simulink model "F16_6DOF_R2024b"  (R2024b)
settings: Solver=VariableStepAuto  StartTime=0.0  StopTime=10.0  RelTol=1e-3
values from neighbouring files (symbols this model uses):
  AeroBP = f16_AerodynamicData.BP    [init_F16.m]
  AeroData = f16_AerodynamicData.data    [init_F16.m]
  b = 30.0 * ft2m    (= 9.144)    [init_F16.m]    (also in trim_F16.m = sin(phi)*sin(beta) + cos(phi)*sin(alpha)*cos(beta))
  cbar = 11.32 * ft2m    (= 3.450336)    [init_F16.m]
  dP_BP = [-100, 25, 50, 100]    [init_F16.m]
  EngBP = f16_EngineData.BP    [init_F16.m]
  EngData = f16_EngineData.data.Thrust_lbs    [init_F16.m]
  Euler_0 = [0;0;0]    [init_F16.m]
  ft2m = 0.3048    [init_F16.m]
  gamma_R_SI = 1.4 * 1716.3 * R_conv    (= 401.812708631)    [init_F16.m]
  h_trop_SI = 35000 * ft2m    (= 10668)    [init_F16.m]
  He = 160.0 * slugft2_to_kgm2    (= 216.930890496)    [init_F16.m]
  I_mat = [ Ixx,  0,   -Ixz ... (first row only)    [init_F16.m]
  inv_I = inv(I_mat)    [init_F16.m]
  inv_tauT_tab = [1.0, 1.0, 0.1, 0.1]    [init_F16.m]
  lapse_SI = 0.703e-5 / ft2m    (= 2.30643044619e-05)    [init_F16.m]
  lbf2N = 4.448222    [init_F16.m]
  m = Weight / g    (= 9298.64438927)    [init_F16.m]
  omega_0 = [0;0;0]    [init_F16.m]
  P1_tab = [0, 50, 100]    [init_F16.m]
  P3_0 = 0    [init_F16.m]    (also in test_thrust_table2.m = interp1(thr_BP, P1_tab, cases(i,3)))
  Pos_0 = [0;0;-3048]    [init_F16.m]
  R0_SI = 2.377e-3 * (slug2kg / ft2m^3)    (= 1.22505555728)    [init_F16.m]
  R_ps_SI = 1715 * R_conv    (= 286.79168448)    [init_F16.m]
  S = 300.0 * (ft2m^2)    (= 27.870912)    [init_F16.m]
  T0_SI = 519.0 / 1.8    (= 288.333333333)    [init_F16.m]
  T_iso_SI = 390 / 1.8    (= 216.666666667)    [init_F16.m]
  thr_BP = [0, 77, 100]    [init_F16.m]
  V_body_0 = [131.28; 0; 0]    [init_F16.m]
  Weight = 20500.0 * lbf2N    (= 91188.551)    [init_F16.m]
  xcg = 0.35    [init_F16.m]
  xcgr = 0.35    [init_F16.m]
libraries: simulink_extras x2
(part 1 of 2)
settings Model: Creator=dilan  LastModifiedBy=emirh

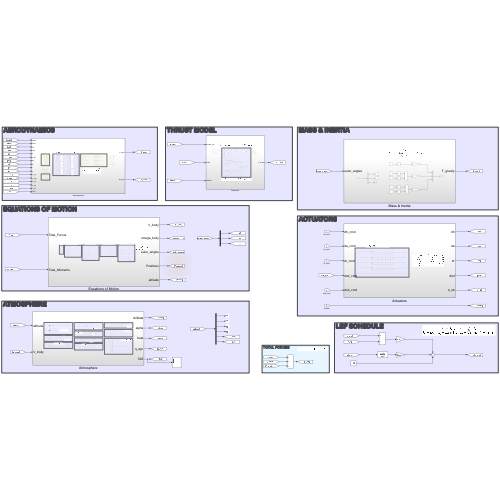
[thumbnail: Simulink's stored preview of the top-level diagram]
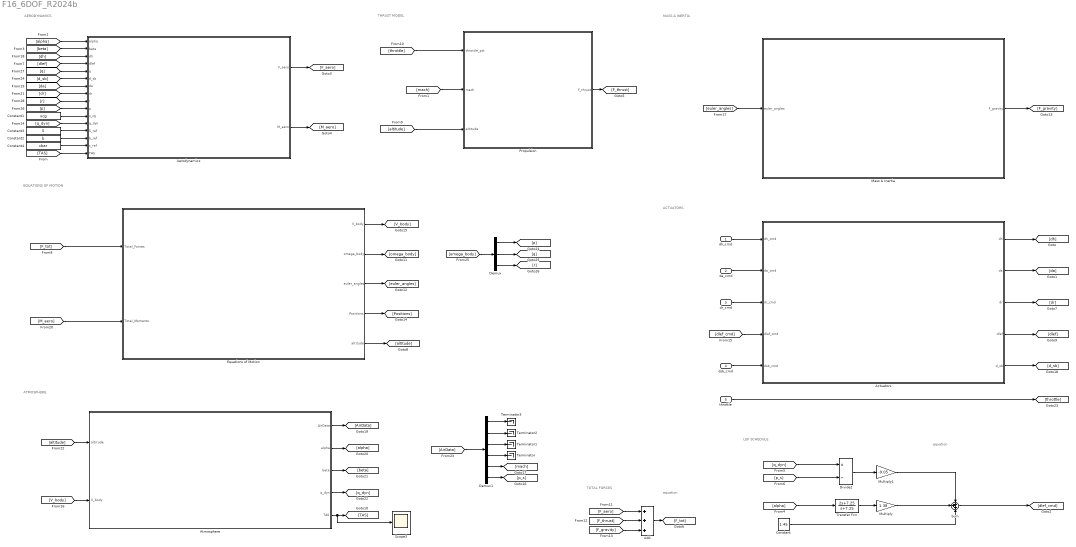
== system F16_6DOF_R2024b ==
  note: TOTAL FORCES
  note: THRUST MODEL
  note: AERODYNAMICS
  note: LEF SCHEDULE
  note: ATMOSPHERE
  note: ACTUATORS
  note: MASS & INERTIA
  note: EQUATIONS OF MOTION
  note: equation
  note: equation
  dh_cmd : Inport
  da_cmd : Inport  Port=2
  dr_cmd : Inport  Port=3
  dsb_cmd : Inport  Port=4
  throttle : Inport  Port=5
  Actuators : Subsystem
  Add : Sum  Inputs=+++
  Aerodynamics : Subsystem
  Atmosphere : Subsystem
  Constant : Constant  Value=1.45
  Constant1 : Constant  Value=xcg
  Constant2 : Constant  Value=b
  Constant3 : Constant  Value=S
  Constant4 : Constant  Value=cbar
  Demux : Demux  Outputs=3
  Demux1 : Demux  Outputs=6
  Divide2 : Product  Inputs=*/
  Equations of Motion : Subsystem
  Mass & Inertia : Subsystem
  Multiply : Gain  Gain=1.38
  Multiply1 : Gain  Gain=-9.05
  Propulsion : Subsystem
  Scope3 : Scope
  Sum : Sum  Inputs=+++
  Terminator{,1..3} (4 alike) : Terminator
  Transfer Fcn : TransferFcn  Numerator=[2 7.25]  Denominator=[1 7.25]
  wires:
  [alpha] -> Aerodynamics/1(alpha)
  [beta] -> Aerodynamics/2(beta)
  Constant/1 -> Sum/3
  Multiply/1 -> Sum/2
  Multiply1/1 -> Sum/1
  Divide2/1 -> Multiply1/1
  Transfer Fcn/1 -> Multiply/1
  [alpha] -> Transfer Fcn/1
  [q_dyn] -> Divide2/1
  [p_s] -> Divide2/2
  [dlef] -> Aerodynamics/4(dlef)
  Aerodynamics/1(F_aero) -> [F_aero]
  Aerodynamics/2(M_aero) -> [M_aero]
  [altitude] -> Propulsion/3(altitude)
  [throttle] -> Propulsion/1(throttle_pct)
  Propulsion/1(F_thrust) -> [F_thrust]
  [F_aero] -> Add/1
  [F_thrust] -> Add/2
  [F_gravity] -> Add/3
  Add/1 -> [F_tot]
  [mach] -> Propulsion/2(mach)
  [q_dyn] -> Aerodynamics/12(q_dyn)
  [altitude] -> Atmosphere/1(altitude)
  [V_body] -> Atmosphere/2(V_body)
  Atmosphere/1(AirData) -> [AirData]
  Atmosphere/2(alpha) -> [alpha]
  Atmosphere/3(beta) -> [beta]
  Atmosphere/4(q_dyn) -> [q_dyn]
  Atmosphere/5(TAS) -> [TAS], Scope3/1
  [AirData] -> Demux1/1
  Demux1/1 -> Terminator3/1
  Demux1/2 -> Terminator2/1
  Demux1/3 -> Terminator1/1
  Demux1/4 -> Terminator/1
  Demux1/5 -> [mach]
  Demux1/6 -> [p_s]
  Sum/1 -> [dlef_cmd]
  dh_cmd/1 -> Actuators/1(dh_cmd)
  Actuators/1(dh) -> [dh]
  da_cmd/1 -> Actuators/2(da_cmd)
  Actuators/2(da) -> [da]
  dr_cmd/1 -> Actuators/3(dr_cmd)
  Actuators/3(dr) -> [dr]
  [dlef_cmd] -> Actuators/4(dlef_cmd)
  Actuators/4(dlef) -> [dlef]
  dsb_cmd/1 -> Actuators/5(dsb_cmd)
  Actuators/5(d_sb) -> [d_sb]
  throttle/1 -> [throttle]
  [dh] -> Aerodynamics/3(dh)
  [da] -> Aerodynamics/7(da)
  [dr] -> Aerodynamics/8(dr)
  [d_sb] -> Aerodynamics/6(d_sb)
  [TAS] -> Aerodynamics/16(TAS)
  [p] -> Aerodynamics/10(p)
  [q] -> Aerodynamics/5(q)
  [r] -> Aerodynamics/9(r)
  Constant1/1 -> Aerodynamics/11(x_cg)
  Constant3/1 -> Aerodynamics/13(S_ref)
  Constant2/1 -> Aerodynamics/14(b_ref)
  Constant4/1 -> Aerodynamics/15(c_ref)
  [euler_angles] -> Mass & Inertia/1(euler_angles)
  Mass & Inertia/1(F_gravity) -> [F_gravity]
  [F_tot] -> Equations of Motion/1(Total_Forces)
  [M_aero] -> Equations of Motion/2(Total_Moments)
  Equations of Motion/1(V_body) -> [V_body]
  Equations of Motion/2(omega_body) -> [omega_body]
  Equations of Motion/3(euler_angles) -> [euler_angles]
  Equations of Motion/4(Positions) -> [Positions]
  Equations of Motion/5(altitude) -> [altitude]
  [omega_body] -> Demux/1
  Demux/1 -> [p]
  Demux/2 -> [q]
  Demux/3 -> [r]

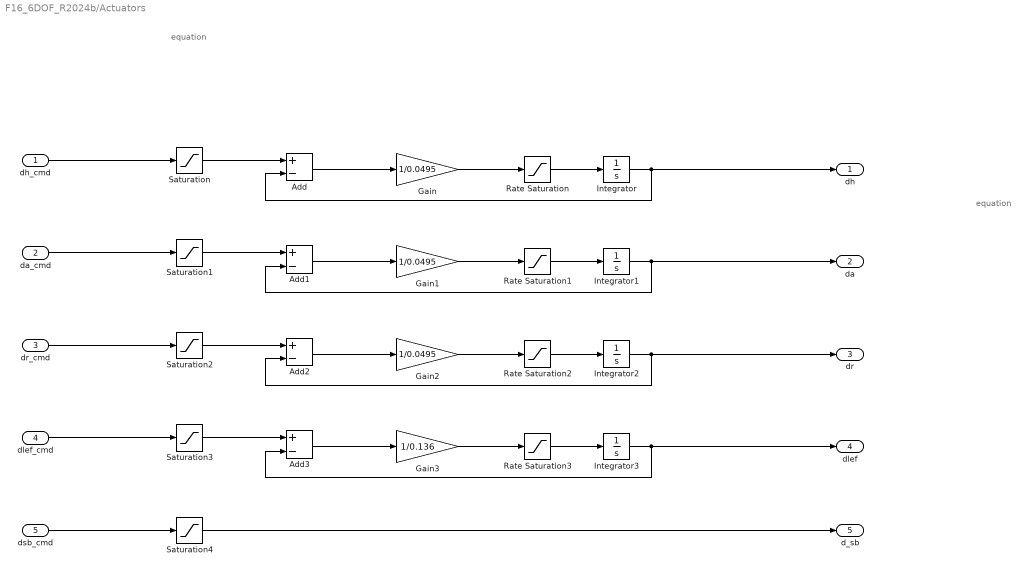
== system F16_6DOF_R2024b/Actuators ==
  note: equation
  note: equation
  dh_cmd : Inport
  da_cmd : Inport  Port=2
  dr_cmd : Inport  Port=3
  dlef_cmd : Inport  Port=4
  dsb_cmd : Inport  Port=5
  Add{,1..3} (4 alike) : Sum  Inputs=+-
  Gain : Gain  Gain=1/0.0495
  Gain1 : Gain  Gain=1/0.0495
  Gain2 : Gain  Gain=1/0.0495
  Gain3 : Gain  Gain=1/0.136
  Integrator{,1..3} (4 alike) : Integrator
  Rate Saturation : Saturate  UpperLimit=60  LowerLimit=-60
  Rate Saturation1 : Saturate  UpperLimit=80  LowerLimit=-80
  Rate Saturation2 : Saturate  UpperLimit=120  LowerLimit=-120
  Rate Saturation3 : Saturate  UpperLimit=25  LowerLimit=-25
  Saturation : Saturate  UpperLimit=25  LowerLimit=-25
  Saturation1 : Saturate  UpperLimit=21.5  LowerLimit=-21.5
  Saturation2 : Saturate  UpperLimit=30  LowerLimit=-30
  Saturation3 : Saturate  UpperLimit=25  LowerLimit=0
  Saturation4 : Saturate  UpperLimit=60  LowerLimit=0
  dh : Outport
  da : Outport  Port=2
  dr : Outport  Port=3
  dlef : Outport  Port=4
  d_sb : Outport  Port=5
  wires:
  dh_cmd/1 -> Saturation/1
  da_cmd/1 -> Saturation1/1
  dr_cmd/1 -> Saturation2/1
  dlef_cmd/1 -> Saturation3/1
  dsb_cmd/1 -> Saturation4/1
  Saturation/1 -> Add/1
  Add/1 -> Gain/1
  Gain/1 -> Rate Saturation/1
  Rate Saturation/1 -> Integrator/1
  Integrator/1 -> dh/1, Add/2
  Integrator1/1 -> da/1, Add1/2
  Rate Saturation1/1 -> Integrator1/1
  Gain1/1 -> Rate Saturation1/1
  Add1/1 -> Gain1/1
  Saturation1/1 -> Add1/1
  Add2/1 -> Gain2/1
  Gain2/1 -> Rate Saturation2/1
  Rate Saturation2/1 -> Integrator2/1
  Integrator2/1 -> dr/1, Add2/2
  Integrator3/1 -> dlef/1, Add3/2
  Rate Saturation3/1 -> Integrator3/1
  Gain3/1 -> Rate Saturation3/1
  Add3/1 -> Gain3/1
  Saturation4/1 -> d_sb/1
  Saturation2/1 -> Add2/1
  Saturation3/1 -> Add3/1

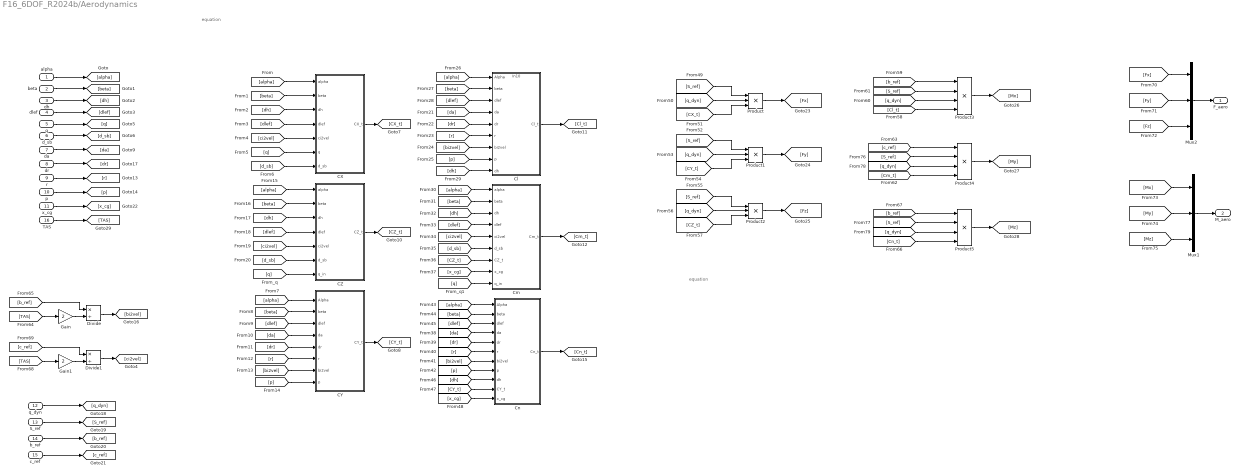
== system F16_6DOF_R2024b/Aerodynamics ==
  note: equation
  note: equation
  alpha : Inport
  beta : Inport  Port=2
  dh : Inport  Port=3
  dlef : Inport  Port=4
  q : Inport  Port=5
  d_sb : Inport  Port=6
  da : Inport  Port=7
  dr : Inport  Port=8
  r : Inport  Port=9
  p : Inport  Port=10
  x_cg : Inport  Port=11
  q_dyn : Inport  Port=12
  S_ref : Inport  Port=13
  b_ref : Inport  Port=14
  c_ref : Inport  Port=15
  TAS : Inport  Port=16
  CX : Subsystem
  CY : Subsystem
  CZ : Subsystem
  Cl : Subsystem
      settings: PortSchema="{\"entries\":[{\"content\":{\"sides\":[{\"content\":{\"connectorIds\":[\"In1\",\"In2\",\"In3\",\"In4\",\"In5\",\"In6\",\"In7\",\"In8\",\"In9\"]},\"type\":\"ConnectorPlacement.EquallySpacedRectSide\",\"uuid\":\"21997383-d6a2-4283-9afe-3717b1097433\"},{\"content\":{\"connectorIds\":[\"Out1\"],\"side\":\"RIGHT\"},\"type\":\"ConnectorPlacement.EquallySpacedRectSide\",\"uuid\":\"dad54f1b-8e4a-4bdd-ae1b-a5d035dab541\"},{\"content\":{\"connectorIds\":[\"In10\"],\"side\":\"TOP\"},\"type\":\"ConnectorPlacement.EquallySpacedRectSide\",\"uuid\":\"167dcd83-ef9f-4972-849f-adf1f6d78b80\"}]},\"type\":\"ConnectorPlacement.EquallySpacedConnector\",\"uuid\":\"1257b268-e5da-46f6-bd8b-58a49b5f7559\"}],\"packageUris\":[\"http://schema.mathworks.com/mf0/Connector/R2020b\"],\"version\":\"1.0\"}"
  Cm : Subsystem
  Cn : Subsystem
  Divide : Product  Inputs=*/
  Divide1 : Product  Inputs=*/
  Gain : Gain  Gain=2
  Gain1 : Gain  Gain=2
  Mux1 : Mux  Inputs=3
  Mux2 : Mux  Inputs=3
  Product : Product  Inputs=3
  Product1 : Product  Inputs=3
  Product2 : Product  Inputs=3
  Product3 : Product  Inputs=4
  Product4 : Product  Inputs=4
  Product5 : Product  Inputs=4
  F_aero : Outport
  M_aero : Outport  Port=2
  wires:
  [c_ref] -> Product4/1
  [dlef] -> CZ/4(dlef)
  [r] -> CY/6(r)
  [beta] -> CY/2(beta)
  [d_sb] -> CX/7(d_sb)
  da/1 -> [da]
  CX/1(CX_t) -> [CX_t]
  q/1 -> [q]
  [dr] -> Cl/5(dr)
  [p] -> CY/8(p)
  dr/1 -> [dr]
  [q_dyn] -> Product3/3
  CZ/1(CZ_t) -> [CZ_t]
  [dr] -> Cn/5(dr)
  [bi2vel] -> Cn/7(bi2vel)
  [da] -> CY/4(da)
  [x_cg] -> Cn/11(x_cg)
  [ci2vel] -> CZ/5(ci2vel)
  Cn/1(Cn_t) -> [Cn_t]
  [alpha] -> CY/1(Alpha)
  CY/1(CY_t) -> [CY_t]
  [Cn_t] -> Product5/4
  [dr] -> CY/5(dr)
  [dlef] -> CY/3(dlef)
  [bi2vel] -> CY/7(bi2vel)
  [q] -> CX/6(q)
  [da] -> Cn/4(da)
  [da] -> Cl/4(da)
  [CY_t] -> Cn/10(CY_t)
  S_ref/1 -> [S_ref]
  [dh] -> Cm/3(dh)
  [My] -> Mux1/2
  [dlef] -> CX/4(dlef)
  p/1 -> [p]
  dh/1 -> [dh]
  alpha/1 -> [alpha]
  Product3/1 -> [Mx]
  [d_sb] -> Cm/6(d_sb)
  [beta] -> CZ/2(beta)
  [ci2vel] -> CX/5(ci2vel)
  beta/1 -> [beta]
  [alpha] -> CX/1(alpha)
  [S_ref] -> Product1/1
  [S_ref] -> Product3/2
  [bi2vel] -> Cl/7(bi2vel)
  [dh] -> CX/3(dh)
  [CZ_t] -> Product2/3
  x_cg/1 -> [x_cg]
  [dlef] -> Cn/3(dlef)
  [Mz] -> Mux1/3
  [dh] -> Cl/9(dh)
  dlef/1 -> [dlef]
  r/1 -> [r]
  d_sb/1 -> [d_sb]
  [beta] -> CX/2(beta)
  [p] -> Cn/8(p)
  b_ref/1 -> [b_ref]
  [dlef] -> Cl/3(dlef)
  [ci2vel] -> Cm/5(ci2vel)
  [r] -> Cl/6(r)
  [r] -> Cn/6(r)
  [p] -> Cl/8(p)
  [d_sb] -> CZ/6(d_sb)
  [dlef] -> Cm/4(dlef)
  Cl/1(Cl_t) -> [Cl_t]
  Product1/1 -> [Fy]
  [dh] -> CZ/3(dh)
  [alpha] -> CZ/1(alpha)
  Product5/1 -> [Mz]
  [b_ref] -> Product5/1
  [alpha] -> Cl/1(Alpha)
  [beta] -> Cl/2(beta)
  q_dyn/1 -> [q_dyn]
  [beta] -> Cm/2(beta)
  [alpha] -> Cm/1(alpha)
  [dh] -> Cn/9(dh)
  [Fx] -> Mux2/1
  [Cm_t] -> Product4/4
  Product4/1 -> [My]
  Cm/1(Cm_t) -> [Cm_t]
  Mux1/1 -> M_aero/1
  [Fz] -> Mux2/3
  Mux2/1 -> F_aero/1
  [Fy] -> Mux2/2
  [Mx] -> Mux1/1
  [beta] -> Cn/2(beta)
  [alpha] -> Cn/1(Alpha)
  c_ref/1 -> [c_ref]
  [Cl_t] -> Product3/4
  [b_ref] -> Product3/1
  [x_cg] -> Cm/8(x_cg)
  [CZ_t] -> Cm/7(CZ_t)
  [q_dyn] -> Product/2
  Product2/1 -> [Fz]
  [S_ref] -> Product/1
  [q_dyn] -> Product1/2
  Product/1 -> [Fx]
  [CX_t] -> Product/3
  [S_ref] -> Product2/1
  [CY_t] -> Product1/3
  [q_dyn] -> Product2/2
  TAS/1 -> [TAS]
  [TAS] -> Gain/1
  Gain/1 -> Divide/2
  [b_ref] -> Divide/1
  Divide/1 -> [bi2vel]
  [c_ref] -> Divide1/1
  Gain1/1 -> Divide1/2
  [TAS] -> Gain1/1
  Divide1/1 -> [ci2vel]
  [q] -> CZ/7(q_in)
  [q] -> Cm/9(q_in)
  [S_ref] -> Product4/2
  [S_ref] -> Product5/2
  [q_dyn] -> Product4/3
  [q_dyn] -> Product5/3

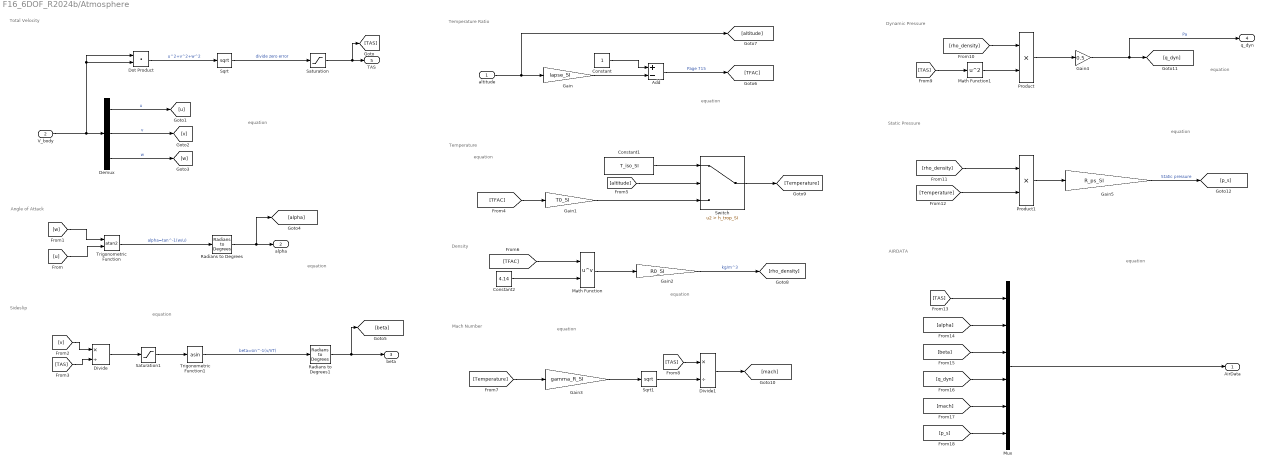
== system F16_6DOF_R2024b/Atmosphere ==
  note: AIRDATA
  note: Static Pressure
  note: Dynamic Pressure
  note: Mach Number
  note: Density
  note: Temperature
  note: Temperature Ratio
  note: Sideslip
  note: Angle of Attack
  note: Total Velocity
  note: equation
  note: equation
  note: equation
  note: equation
  note: equation
  note: equation
  note: equation
  note: equation
  note: equation
  note: equation
  altitude : Inport
  V_body : Inport  Port=2
  Add : Sum  Inputs=+-
  Constant : Constant
  Constant1 : Constant  Value=T_iso_SI
  Constant2 : Constant  Value=4.14
  Demux : Demux  Outputs=3
  Divide : Product  Inputs=*/
  Divide1 : Product  Inputs=*/
  Dot Product : DotProduct  OutDataTypeStr=Inherit: Inherit via internal rule
  Gain : Gain  Gain=lapse_SI
  Gain1 : Gain  Gain=T0_SI
  Gain2 : Gain  Gain=R0_SI
  Gain3 : Gain  Gain=gamma_R_SI
  Gain4 : Gain  Gain=0.5
  Gain5 : Gain  Gain=R_ps_SI
  Math Function : Math  Operator=pow
  Math Function1 : Math  Operator=square
  Mux : Mux  Inputs=6
  Product : Product
  Product1 : Product
  Radians to Degrees : simulink_extras/Transformations/Radians to Degrees
  Radians to Degrees1 : simulink_extras/Transformations/Radians to Degrees
  Saturation : Saturate  UpperLimit=inf  LowerLimit=0.1
  Saturation1 : Saturate  UpperLimit=1  LowerLimit=-1
  Sqrt : Sqrt
  Sqrt1 : Sqrt
  Switch : Switch  Criteria=u2 > Threshold  Threshold=h_trop_SI  SaturateOnIntegerOverflow=off  InputSameDT=off
  Trigonometric Function : Trigonometry  Operator=atan2
  Trigonometric Function1 : Trigonometry  Operator=asin
  AirData : Outport
  alpha : Outport  Port=2
  beta : Outport  Port=3
  q_dyn : Outport  Port=4
  TAS : Outport  Port=5
  wires:
  V_body/1 -> Dot Product/2, Dot Product/1, Demux/1
  altitude/1 -> [altitude], Gain/1
  Dot Product/1 -> Sqrt/1  "u^2+v^2+w^2"
  Demux/1 -> [u]  "u"
  Demux/2 -> [v]  "v"
  Demux/3 -> [w]  "w"
  Sqrt/1 -> Saturation/1  "divide zero error"
  Saturation/1 -> [TAS], TAS/1
  [w] -> Trigonometric Function/1
  [u] -> Trigonometric Function/2
  Trigonometric Function/1 -> Radians to Degrees/1  "alpha=tan^-1(w/u)"
  Radians to Degrees/1 -> [alpha], alpha/1
  [v] -> Divide/1
  [TAS] -> Divide/2
  Divide/1 -> Saturation1/1
  Saturation1/1 -> Trigonometric Function1/1
  Trigonometric Function1/1 -> Radians to Degrees1/1  "beta=sin^-1(v/VT)"
  Radians to Degrees1/1 -> [beta], beta/1
  Constant/1 -> Add/1
  Gain/1 -> Add/2
  Add/1 -> [TFAC]  "Page 715"
  [TFAC] -> Gain1/1
  Constant1/1 -> Switch/1
  [altitude] -> Switch/2
  Gain1/1 -> Switch/3
  [TFAC] -> Math Function/1
  Constant2/1 -> Math Function/2
  Math Function/1 -> Gain2/1
  Gain2/1 -> [rho_density]  "kg/m^3"
  Switch/1 -> [Temperature]
  [Temperature] -> Gain3/1
  Gain3/1 -> Sqrt1/1
  Sqrt1/1 -> Divide1/2
  [TAS] -> Divide1/1
  Divide1/1 -> [mach]
  [TAS] -> Math Function1/1
  [rho_density] -> Product/1
  Math Function1/1 -> Product/2
  Product/1 -> Gain4/1
  Gain4/1 -> q_dyn/1, [q_dyn]  "Pa"
  [rho_density] -> Product1/1
  [Temperature] -> Product1/2
  Product1/1 -> Gain5/1
  Gain5/1 -> [p_s]  "Static pressure"
  [TAS] -> Mux/1
  [alpha] -> Mux/2
  [beta] -> Mux/3
  [q_dyn] -> Mux/4
  [mach] -> Mux/5
  [p_s] -> Mux/6
  Mux/1 -> AirData/1

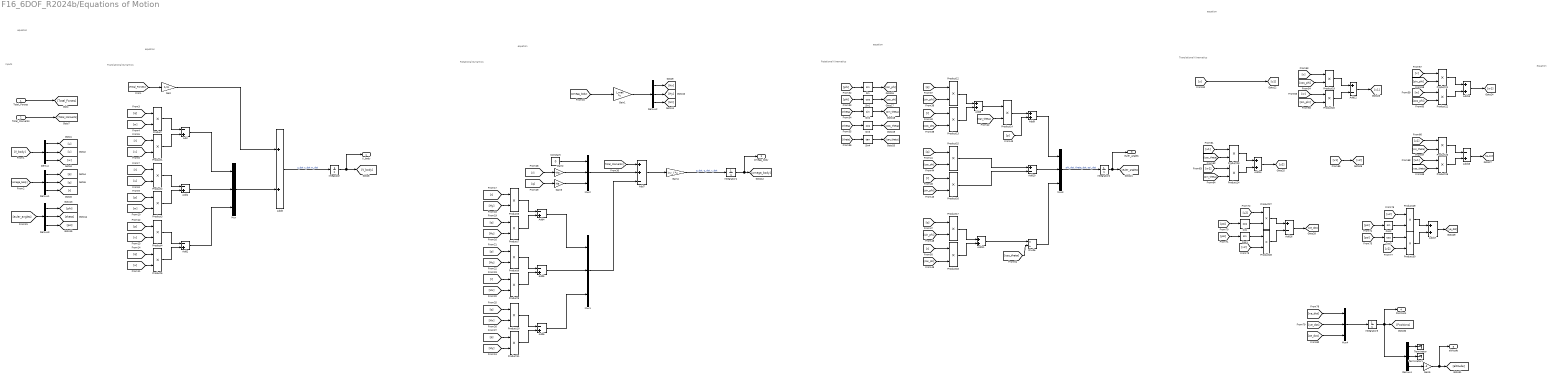
== system F16_6DOF_R2024b/Equations of Motion ==
  note: Inputs
  note: Translational Kinematics
  note: Rotational Kinematics
  note: Rotational Dynamics
  note: Translational Dynamics
  note: equation
  note: equation
  note: equation
  note: equation
  note: equation
  note: equation
  Total_Forces : Inport
  Total_Moments : Inport  Port=2
  Add{,1..2,4..6,15} (7 alike) : Sum  Inputs=-+
  Add10 : Sum  Inputs=+-
  Add{3,8..9,11,13..14,17} (7 alike) : Sum
  Add12 : Sum  Inputs=+-
  Add16 : Sum  Inputs=+-
  Add7 : Sum  Inputs=++-
  Constant : Constant  Value=0
  Cos : Trigonometry  Operator=cos
  Cos1 : Trigonometry
  Cos2 : Trigonometry
  Cos3 : Trigonometry  Operator=cos
  Demux{,1..4} (5 alike) : Demux  Outputs=3
  Divide : Product  Inputs=*/
  Gain : Gain  Gain=1/m
  Gain1 : Gain  Gain=I_mat  Multiplication=Matrix(K*u)
  Gain2 : Gain  Gain=-He
  Gain3 : Gain  Gain=He
  Gain4 : Gain  Gain=inv_I  Multiplication=Matrix(K*u)
  Gain5 : Gain  Gain=-1
  Integrator : Integrator  InitialCondition=V_body_0
  Integrator1 : Integrator  InitialCondition=omega_0
  Integrator2 : Integrator  InitialCondition=Euler_0
  Integrator3 : Integrator  InitialCondition=Pos_0
  Mux{,1..4} (5 alike) : Mux  Inputs=3
  Product{,1..30} (31 alike) : Product
  Sin : Trigonometry
  Sin1 : Trigonometry  Operator=cos
  Sin2 : Trigonometry
  Sin3 : Trigonometry  Operator=cos
  Sin4 : Trigonometry  Operator=tan
  Terminator : Terminator
  Terminator1 : Terminator
  V_body : Outport
  omega_body : Outport  Port=2
  euler_angles : Outport  Port=3
  Positions : Outport  Port=4
  altitude : Outport  Port=5
  wires:
  Total_Forces/1 -> [Total_Forces]
  [Total_Forces] -> Gain/1
  [V_body] -> Demux/1
  [omega_body] -> Demux1/1
  Demux/1 -> [u]
  Demux/2 -> [v]
  Demux/3 -> [w]
  Demux1/1 -> [p]
  Demux1/2 -> [q]
  Demux1/3 -> [r]
  [q] -> Product/1
  [w] -> Product/2
  [v] -> Product1/2
  [r] -> Product1/1
  Product/1 -> Add/1
  Product1/1 -> Add/2
  Product3/1 -> Add1/2
  Product2/1 -> Add1/1
  [p] -> Product3/1
  [w] -> Product3/2
  [u] -> Product2/2
  [r] -> Product2/1
  [p] -> Product4/1
  [v] -> Product4/2
  [u] -> Product5/2
  [q] -> Product5/1
  Product4/1 -> Add2/1
  Product5/1 -> Add2/2
  Add1/1 -> Mux/2
  Add/1 -> Mux/1
  Add2/1 -> Mux/3
  Mux/1 -> Add3/2
  Gain/1 -> Add3/1
  Total_Moments/1 -> [Total_Moments]
  Add3/1 -> Integrator/1  "u_dot v_dot w_dot"
  Integrator/1 -> V_body/1, [V_body]
  [omega_body] -> Gain1/1
  Gain1/1 -> Demux2/1
  Demux2/3 -> [Hz]
  Demux2/2 -> [Hy]
  Demux2/1 -> [Hx]
  Product7/1 -> Add4/2
  Product6/1 -> Add4/1
  [q] -> Product7/1
  [Hz] -> Product7/2
  [Hy] -> Product6/2
  [r] -> Product6/1
  [p] -> Product8/1
  [Hz] -> Product8/2
  [Hx] -> Product9/2
  [r] -> Product9/1
  Product8/1 -> Add5/1
  Product9/1 -> Add5/2
  Product11/1 -> Add6/2
  Product10/1 -> Add6/1
  [p] -> Product11/1
  [Hy] -> Product11/2
  [Hx] -> Product10/2
  [q] -> Product10/1
  Add5/1 -> Mux1/2
  Add4/1 -> Mux1/1
  Add6/1 -> Mux1/3
  Constant/1 -> Mux2/1
  [r] -> Gain2/1
  Gain2/1 -> Mux2/2
  Gain3/1 -> Mux2/3
  [q] -> Gain3/1
  [Total_Moments] -> Add7/1
  Mux2/1 -> Add7/2
  Mux1/1 -> Add7/3
  Add7/1 -> Gain4/1
  Gain4/1 -> Integrator1/1  "p_dot, q_dot, r_dot"
  Integrator1/1 -> omega_body/1, [omega_body]
  [euler_angles] -> Demux3/1
  Demux3/1 -> [phi]
  Demux3/2 -> [theta]
  Demux3/3 -> [psi]
  Sin1/1 -> [cos_phi]
  Sin/1 -> [sin_phi]
  Sin4/1 -> [tan_theta]
  [phi] -> Sin/1
  [theta] -> Sin3/1
  Sin2/1 -> [sin_theta]
  Sin3/1 -> [cos_theta]
  [theta] -> Sin2/1
  [phi] -> Sin1/1
  [theta] -> Sin4/1
  [q] -> Product12/1
  [sin_phi] -> Product12/2
  [r] -> Product13/1
  [cos_phi] -> Product13/2
  Product12/1 -> Add8/1
  Product13/1 -> Add8/2
  [tan_theta] -> Product14/2
  Add8/1 -> Product14/1
  Product14/1 -> Add9/1
  [p] -> Add9/2
  [sin_phi] -> Product16/2
  [r] -> Product16/1
  [cos_phi] -> Product15/2
  [q] -> Product15/1
  [q] -> Product17/1
  [sin_phi] -> Product17/2
  [r] -> Product18/1
  [cos_phi] -> Product18/2
  Product17/1 -> Add11/1
  Product15/1 -> Add10/1
  Product16/1 -> Add10/2
  Product18/1 -> Add11/2
  Add11/1 -> Divide/1
  [cos_theta] -> Divide/2
  Add9/1 -> Mux3/1
  Add10/1 -> Mux3/2
  Divide/1 -> Mux3/3
  Mux3/1 -> Integrator2/1  "phi_dot, theta_dot, psi_dot"
  Integrator2/1 -> euler_angles/1, [euler_angles]
  [u] -> [u1]
  [v] -> Product19/1
  [cos_phi] -> Product19/2
  [sin_phi] -> Product20/2
  [w] -> Product20/1
  Product20/1 -> Add12/2
  Product19/1 -> Add12/1
  Add12/1 -> [v1]
  Product21/1 -> Add13/1
  Product22/1 -> Add13/2
  [w] -> Product22/1
  [cos_phi] -> Product22/2
  [sin_phi] -> Product21/2
  [v] -> Product21/1
  Add13/1 -> [w1]
  [u1] -> Product23/1
  [cos_theta] -> Product23/2
  [sin_theta] -> Product24/2
  [w1] -> Product24/1
  Product24/1 -> Add14/2
  Product23/1 -> Add14/1
  Add14/1 -> [u2]
  [v1] -> [v2]
  Add15/1 -> [ze_dot]
  Product25/1 -> Add15/1
  Product26/1 -> Add15/2
  [w1] -> Product26/1
  [cos_theta] -> Product26/2
  [sin_theta] -> Product25/2
  [u1] -> Product25/1
  [psi] -> Cos/1
  [psi] -> Cos1/1
  [u2] -> Product27/1
  Cos/1 -> Product27/2
  Cos1/1 -> Product28/1
  [v2] -> Product28/2
  Product28/1 -> Add16/2
  Product27/1 -> Add16/1
  Add16/1 -> [xe_dot]
  Add17/1 -> [ye_dot]
  Product29/1 -> Add17/1
  Product30/1 -> Add17/2
  [v2] -> Product30/2
  Cos3/1 -> Product30/1
  Cos2/1 -> Product29/2
  [u2] -> Product29/1
  [psi] -> Cos3/1
  [psi] -> Cos2/1
  [ye_dot] -> Mux4/2
  [xe_dot] -> Mux4/1
  [ze_dot] -> Mux4/3
  Mux4/1 -> Integrator3/1
  Integrator3/1 -> Demux4/1, Positions/1, [Positions]
  Demux4/1 -> Terminator/1
  Demux4/2 -> Terminator1/1
  Demux4/3 -> Gain5/1
  Gain5/1 -> altitude/1, [altitude]

== system F16_6DOF_R2024b/Mass & Inertia ==
  note: equation
  euler_angles : Inport
  Cos : Trigonometry  Operator=cos
  Cos1 : Trigonometry  Operator=cos
  Cos2 : Trigonometry  Operator=cos
  Demux : Demux  Outputs=3
  Gain : Gain  Gain=-Weight
  Gain1 : Gain  Gain=Weight
  Gain2 : Gain  Gain=Weight
  Mux : Mux  Inputs=3
  Product : Product
  Product1 : Product
  Sin : Trigonometry
  Sin1 : Trigonometry
  Terminator : Terminator
  F_gravity : Outport
  wires:
  euler_angles/1 -> Demux/1
  Demux/1 -> [phi]
  Demux/2 -> [theta]
  [theta] -> Sin/1
  [theta] -> Cos/1
  Sin/1 -> Gain/1
  Cos/1 -> Product/1
  [phi] -> Sin1/1
  Sin1/1 -> Product/2
  Product/1 -> Gain1/1
  [theta] -> Cos1/1
  Cos1/1 -> Product1/1
  [phi] -> Cos2/1
  Cos2/1 -> Product1/2
  Product1/1 -> Gain2/1
  Mux/1 -> F_gravity/1
  Gain/1 -> Mux/1
  Gain1/1 -> Mux/2
  Gain2/1 -> Mux/3
  Demux/3 -> Terminator/1

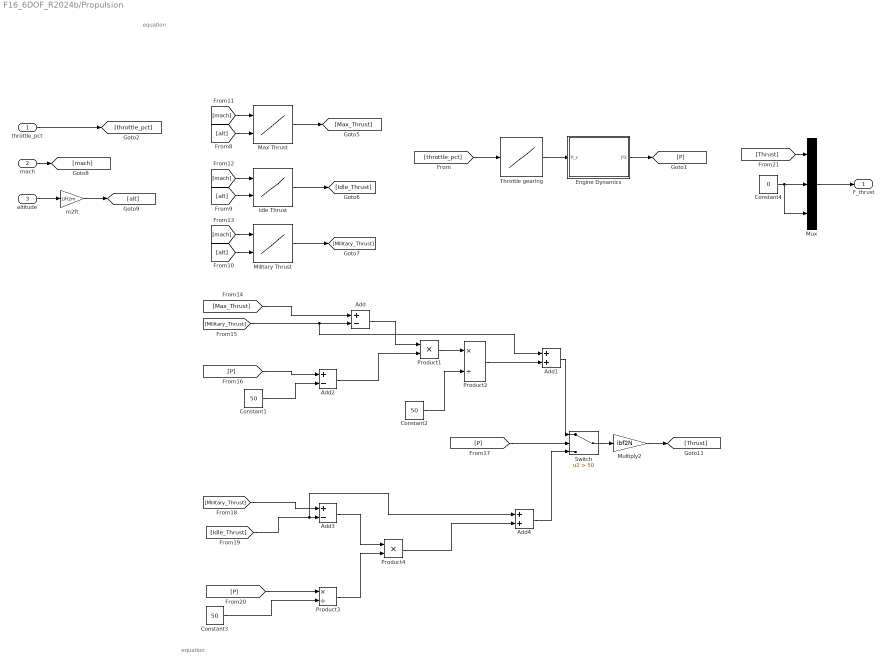
== system F16_6DOF_R2024b/Propulsion ==
  note: equation
  note: equation
  throttle_pct : Inport
  mach : Inport  Port=2
  altitude : Inport  Port=3
  Add : Sum  Inputs=+-
  Add1 : Sum
  Add2 : Sum  Inputs=+-
  Add3 : Sum  Inputs=+-
  Add4 : Sum
  Constant1 : Constant  Value=50
  Constant2 : Constant  Value=50
  Constant3 : Constant  Value=50
  Constant4 : Constant  Value=0
  Engine Dynamics : Subsystem
  Idle Thrust : Lookup_n-D  BreakpointsForDimension1=EngBP.idle.mach  BreakpointsForDimension2=EngBP.idle.alt_ft  BreakpointsForDimension3=[5, 7]  Table=EngData.idle  ExtrapMethod=Clip  DiagnosticForOutOfRangeInput=Warning  InternalRulePriority=Speed  RndMeth=Simplest
      settings: InputPortMap=u0,u1
  Max Thrust : Lookup_n-D  BreakpointsForDimension1=EngBP.max.mach  BreakpointsForDimension2=EngBP.max.alt_ft  BreakpointsForDimension3=[5, 7]  Table=EngData.max  ExtrapMethod=Clip  DiagnosticForOutOfRangeInput=Warning  InternalRulePriority=Speed  RndMeth=Simplest
      settings: InputPortMap=u0,u1
  Military Thrust : Lookup_n-D  BreakpointsForDimension1=EngBP.mil.mach  BreakpointsForDimension2=EngBP.mil.alt_ft  BreakpointsForDimension3=[5, 7]  Table=EngData.mil  ExtrapMethod=Clip  DiagnosticForOutOfRangeInput=Warning  InternalRulePriority=Speed  RndMeth=Simplest
      settings: InputPortMap=u0,u1
  Multiply2 : Gain  Gain=lbf2N
  Mux : Mux  Inputs=3
  Product1 : Product
  Product2 : Product  Inputs=*/
  Product3 : Product  Inputs=*/
  Product4 : Product
  Switch : Switch  Criteria=u2 > Threshold  Threshold=50  SaturateOnIntegerOverflow=off  InputSameDT=off
  Throttle gearing : Lookup_n-D  NumberOfTableDimensions=1  BreakpointsForDimension1=thr_BP  Table=P1_tab  ExtrapMethod=Clip  InternalRulePriority=Speed  RndMeth=Simplest
  m2ft : Gain  Gain=1/ft2m
  F_thrust : Outport
  wires:
  [Idle_Thrust] -> Add4/1, Add3/2
  [Thrust] -> Mux/1
  [alt] -> Idle Thrust/2
  Product4/1 -> Add4/2
  [Military_Thrust] -> Add3/1
  mach/1 -> [mach]
  Add4/1 -> Switch/3
  m2ft/1 -> [alt]
  [Military_Thrust] -> Add/2, Add1/1
  [Max_Thrust] -> Add/1
  Product1/1 -> Product2/1
  Idle Thrust/1 -> [Idle_Thrust]
  Product3/1 -> Product4/2
  Add3/1 -> Product4/1
  Constant3/1 -> Product3/2
  [mach] -> Military Thrust/1
  [alt] -> Max Thrust/2
  [mach] -> Max Thrust/1
  Military Thrust/1 -> [Military_Thrust]
  Constant4/1 -> Mux/3, Mux/2
  [mach] -> Idle Thrust/1
  Constant1/1 -> Add2/2
  [alt] -> Military Thrust/2
  Max Thrust/1 -> [Max_Thrust]
  [P] -> Switch/2
  [P] -> Add2/1
  altitude/1 -> m2ft/1
  [P] -> Product3/1
  Switch/1 -> Multiply2/1
  Product2/1 -> Add1/2
  Add2/1 -> Product1/2
  Constant2/1 -> Product2/2
  Add/1 -> Product1/1
  Add1/1 -> Switch/1
  Mux/1 -> F_thrust/1
  Multiply2/1 -> [Thrust]
  throttle_pct/1 -> [throttle_pct]
  Engine Dynamics/1(P3) -> [P]
  Throttle gearing/1 -> Engine Dynamics/1(P_c)
  [throttle_pct] -> Throttle gearing/1

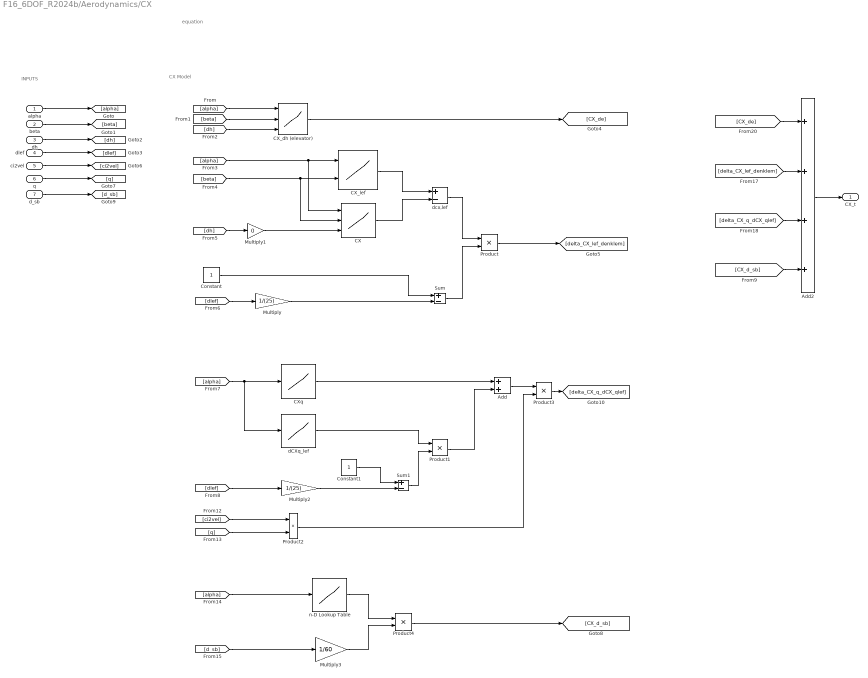
== system F16_6DOF_R2024b/Aerodynamics/CX ==
  note: CX Model
  note: INPUTS
  note: equation
  alpha : Inport
  beta : Inport  Port=2
  dh : Inport  Port=3
  dlef : Inport  Port=4
  ci2vel : Inport  Port=5
  q : Inport  Port=6
  d_sb : Inport  Port=7
  Add : Sum
  Add2 : Sum  Inputs=++++
  CX : Lookup_n-D  NumberOfTableDimensions=3  BreakpointsForDimension1=AeroBP.CX.CX.alpha  BreakpointsForDimension2=AeroBP.CX.CX.beta  BreakpointsForDimension3=AeroBP.CX.CX.dHT  Table=AeroData.CX.CX  ExtrapMethod=Clip  InternalRulePriority=Speed  RndMeth=Simplest
      settings: InputPortMap=u0,u1,u2
  CX_dh (elevator) : Lookup_n-D  NumberOfTableDimensions=3  BreakpointsForDimension1=AeroBP.CX.CX.alpha  BreakpointsForDimension2=AeroBP.CX.CX.beta  BreakpointsForDimension3=AeroBP.CX.CX.dHT  Table=AeroData.CX.CX  ExtrapMethod=Clip  InternalRulePriority=Speed  RndMeth=Simplest
      settings: InputPortMap=u0,u1,u2
  CX_lef : Lookup_n-D  BreakpointsForDimension1=AeroBP.CX.CXlef.alpha  BreakpointsForDimension2=AeroBP.CX.CXlef.beta  BreakpointsForDimension3=[5, 7]  Table=AeroData.CX.CXlef  ExtrapMethod=Clip  InternalRulePriority=Speed  RndMeth=Simplest
      settings: InputPortMap=u0,u1
  CXq : Lookup_n-D  NumberOfTableDimensions=1  BreakpointsForDimension1=AeroBP.CX.CXq.alpha  BreakpointsForDimension3=[5, 7]  Table=AeroData.CX.CXq  ExtrapMethod=Clip  InternalRulePriority=Speed  RndMeth=Simplest
  Constant : Constant
  Constant1 : Constant
  Multiply : Gain  Gain=1/(25)
  Multiply1 : Gain  Gain=0
  Multiply2 : Gain  Gain=1/(25)
  Multiply3 : Gain  Gain=1/60
  Product{,1..4} (5 alike) : Product
  Sum : Sum  Inputs=+-
  Sum1 : Sum  Inputs=+-
  dCXq_lef : Lookup_n-D  NumberOfTableDimensions=1  BreakpointsForDimension1=AeroBP.CX.deltaCXqlef.alpha  BreakpointsForDimension3=[5, 7]  Table=AeroData.CX.deltaCXqlef  ExtrapMethod=Clip  InternalRulePriority=Speed  RndMeth=Simplest
  dcx,lef : Sum  Inputs=+-
  n-D Lookup Table : Lookup_n-D  NumberOfTableDimensions=1  BreakpointsForDimension1=AeroBP.CX.deltaCXSB.alpha  BreakpointsForDimension3=[5, 7]  Table=AeroData.CX.deltaCXSB  ExtrapMethod=Clip  InternalRulePriority=Speed  RndMeth=Simplest
  CX_t : Outport
  wires:
  [alpha] -> CXq/1, dCXq_lef/1
  Add/1 -> Product3/1
  dcx,lef/1 -> Product/1
  [beta] -> CX/2, CX_lef/2
  Product2/1 -> Product3/2
  [alpha] -> n-D Lookup Table/1
  d_sb/1 -> [d_sb]
  [alpha] -> CX/1, CX_lef/1
  q/1 -> [q]
  [beta] -> CX_dh (elevator)/2
  Multiply2/1 -> Sum1/2
  Product3/1 -> [delta_CX_q_dCX_qlef]
  [dlef] -> Multiply/1
  [d_sb] -> Multiply3/1
  CXq/1 -> Add/1
  dCXq_lef/1 -> Product1/1
  Sum/1 -> Product/2
  Product1/1 -> Add/2
  Sum1/1 -> Product1/2
  Product/1 -> [delta_CX_lef_denklem]
  [ci2vel] -> Product2/1
  Constant1/1 -> Sum1/1
  Product4/1 -> [CX_d_sb]
  [dh] -> Multiply1/1
  alpha/1 -> [alpha]
  [alpha] -> CX_dh (elevator)/1
  beta/1 -> [beta]
  CX_lef/1 -> dcx,lef/1
  CX_dh (elevator)/1 -> [CX_de]
  Multiply/1 -> Sum/2
  [dh] -> CX_dh (elevator)/3
  [dlef] -> Multiply2/1
  CX/1 -> dcx,lef/2
  [q] -> Product2/2
  Multiply1/1 -> CX/3
  Constant/1 -> Sum/1
  n-D Lookup Table/1 -> Product4/1
  dlef/1 -> [dlef]
  dh/1 -> [dh]
  ci2vel/1 -> [ci2vel]
  Multiply3/1 -> Product4/2
  [CX_d_sb] -> Add2/4
  [delta_CX_q_dCX_qlef] -> Add2/3
  [delta_CX_lef_denklem] -> Add2/2
  [CX_de] -> Add2/1
  Add2/1 -> CX_t/1

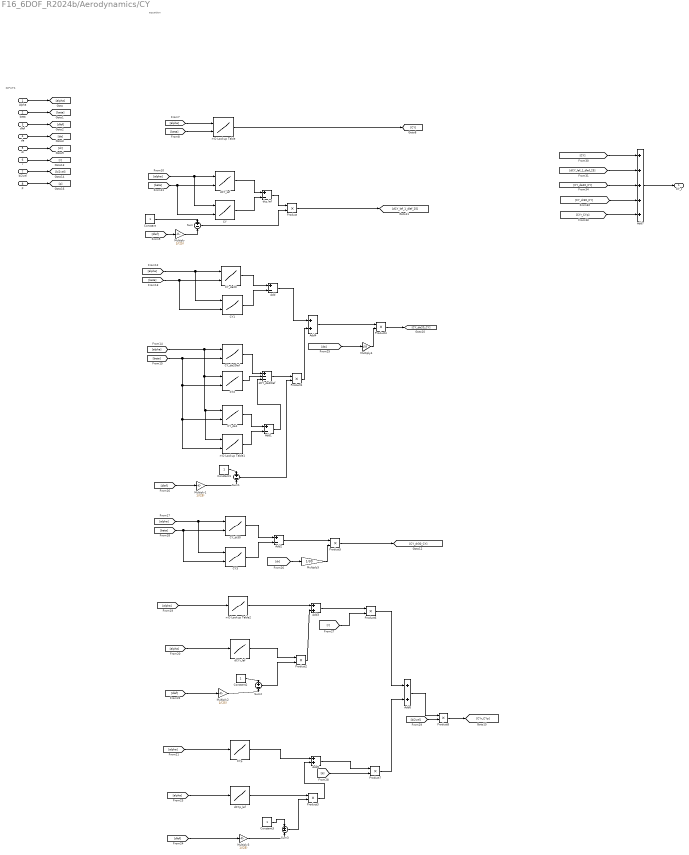
== system F16_6DOF_R2024b/Aerodynamics/CY ==
  note: INPUTS
  note: equation
  Alpha : Inport
  beta : Inport  Port=2
  dlef : Inport  Port=3
  da : Inport  Port=4
  dr : Inport  Port=5
  r : Inport  Port=6
  bi2vel : Inport  Port=7
  p : Inport  Port=8
  Add : Sum  Inputs=+-
  Add1 : Sum  Inputs=+-
  Add2 : Sum  Inputs=+-
  Add{3..6} (4 alike) : Sum
  Add7 : Sum  Inputs=5
  CY : Lookup_n-D  BreakpointsForDimension1=AeroBP.CY.CY.alpha  BreakpointsForDimension2=AeroBP.CY.CY.beta  BreakpointsForDimension3=[5, 7]  Table=AeroData.CY.CY  ExtrapMethod=Clip  InternalRulePriority=Speed  RndMeth=Simplest
      settings: InputPortMap=u0,u1
  CY1 : Lookup_n-D  BreakpointsForDimension1=AeroBP.CY.CY.alpha  BreakpointsForDimension2=AeroBP.CY.CY.beta  BreakpointsForDimension3=[5, 7]  Table=AeroData.CY.CY  ExtrapMethod=Clip  InternalRulePriority=Speed  RndMeth=Simplest
      settings: InputPortMap=u0,u1
  CY2 : Lookup_n-D  BreakpointsForDimension1=AeroBP.CY.CYlef.alpha  BreakpointsForDimension2=AeroBP.CY.CYlef.beta  BreakpointsForDimension3=[5, 7]  Table=AeroData.CY.CYlef  ExtrapMethod=Clip  InternalRulePriority=Speed  RndMeth=Simplest
      settings: InputPortMap=u0,u1
  CY3 : Lookup_n-D  BreakpointsForDimension1=AeroBP.CY.CY.alpha  BreakpointsForDimension2=AeroBP.CY.CY.beta  BreakpointsForDimension3=[5, 7]  Table=AeroData.CY.CY  ExtrapMethod=Clip  InternalRulePriority=Speed  RndMeth=Simplest
      settings: InputPortMap=u0,u1
  CY_da1 : Lookup_n-D  BreakpointsForDimension1=AeroBP.CY.CYda20.alpha  BreakpointsForDimension2=AeroBP.CY.CYda20.beta  BreakpointsForDimension3=[5, 7]  Table=AeroData.CY.CYda20  ExtrapMethod=Clip  InternalRulePriority=Speed  RndMeth=Simplest
      settings: InputPortMap=u0,u1
  CY_da20 : Lookup_n-D  BreakpointsForDimension1=AeroBP.CY.CYda20.alpha  BreakpointsForDimension2=AeroBP.CY.CYda20.beta  BreakpointsForDimension3=[5, 7]  Table=AeroData.CY.CYda20  ExtrapMethod=Clip  InternalRulePriority=Speed  RndMeth=Simplest
      settings: InputPortMap=u0,u1
  CY_da20lef : Lookup_n-D  BreakpointsForDimension1=AeroBP.CY.CYda20lef.alpha  BreakpointsForDimension2=AeroBP.CY.CYda20lef.beta  BreakpointsForDimension3=[5, 7]  Table=AeroData.CY.CYda20lef  ExtrapMethod=Clip  InternalRulePriority=Speed  RndMeth=Simplest
      settings: InputPortMap=u0,u1
  CY_dr30 : Lookup_n-D  BreakpointsForDimension1=AeroBP.CY.CYdr30.alpha  BreakpointsForDimension2=AeroBP.CY.CYdr30.beta  BreakpointsForDimension3=[5, 7]  Table=AeroData.CY.CYdr30  ExtrapMethod=Clip  InternalRulePriority=Speed  RndMeth=Simplest
      settings: InputPortMap=u0,u1
  CYp : Lookup_n-D  NumberOfTableDimensions=1  BreakpointsForDimension1=AeroBP.CY.CYp.alpha  BreakpointsForDimension3=[5, 7]  Table=AeroData.CY.CYp  ExtrapMethod=Clip  InternalRulePriority=Speed  RndMeth=Simplest
  Constant{,1..3} (4 alike) : Constant
  Multiply{,1..3} (4 alike) : Gain  Gain=1/(25)
  Multiply4 : Gain  Gain=1/20
  Multiply5 : Gain  Gain=1/30
  Product{,1..8} (9 alike) : Product
  Sum{,1..3} (4 alike) : Sum  Inputs=+-
  dCY_da20lef : Sum  Inputs=+--
  dCY_lef : Lookup_n-D  BreakpointsForDimension1=AeroBP.CY.CYlef.alpha  BreakpointsForDimension2=AeroBP.CY.CYlef.beta  BreakpointsForDimension3=[5, 7]  Table=AeroData.CY.CYlef  ExtrapMethod=Clip  InternalRulePriority=Speed  RndMeth=Simplest
      settings: InputPortMap=u0,u1
  dCYp_lef : Lookup_n-D  NumberOfTableDimensions=1  BreakpointsForDimension1=AeroBP.CY.deltaCYplef.alpha  BreakpointsForDimension3=[5, 7]  Table=AeroData.CY.deltaCYplef  ExtrapMethod=Clip  InternalRulePriority=Speed  RndMeth=Simplest
  dCYr_lef : Lookup_n-D  NumberOfTableDimensions=1  BreakpointsForDimension1=AeroBP.CY.deltaCYrlef.alpha  BreakpointsForDimension3=[5, 7]  Table=AeroData.CY.deltaCYrlef  ExtrapMethod=Clip  InternalRulePriority=Speed  RndMeth=Simplest
  dcy,lef : Sum  Inputs=+-
  n-D Lookup Table : Lookup_n-D  BreakpointsForDimension1=AeroBP.CY.CY.alpha  BreakpointsForDimension2=AeroBP.CY.CY.beta  BreakpointsForDimension3=[5, 7]  Table=AeroData.CY.CY  ExtrapMethod=Clip  InternalRulePriority=Speed  RndMeth=Simplest
      settings: InputPortMap=u0,u1
  n-D Lookup Table1 : Lookup_n-D  BreakpointsForDimension1=AeroBP.CY.CY.alpha  BreakpointsForDimension2=AeroBP.CY.CY.beta  BreakpointsForDimension3=[5, 7]  Table=AeroData.CY.CY  ExtrapMethod=Clip  InternalRulePriority=Speed  RndMeth=Simplest
      settings: InputPortMap=u0,u1
  n-D Lookup Table2 : Lookup_n-D  NumberOfTableDimensions=1  BreakpointsForDimension1=AeroBP.CY.CYr.alpha  BreakpointsForDimension3=[5, 7]  Table=AeroData.CY.CYr  ExtrapMethod=Clip  InternalRulePriority=Speed  RndMeth=Simplest
  CY_t : Outport
  wires:
  [r] -> Product6/2
  Constant1/1 -> Sum1/1
  dcy,lef/1 -> Product/1
  Product1/1 -> Add4/2
  Add2/1 -> Product5/1
  Constant/1 -> Sum/1
  [alpha] -> n-D Lookup Table1/1, CY_da1/1, CY2/1, CY_da20lef/1
  Sum1/1 -> Product1/2
  Add/1 -> Add4/1
  [alpha] -> CY_da20/1, CY1/1
  [dlef] -> Multiply/1
  [beta] -> CY3/2, CY_dr30/2
  n-D Lookup Table/1 -> [CY]
  Product6/1 -> Add6/1
  [beta] -> CY/2, dCY_lef/2
  n-D Lookup Table2/1 -> Add3/1
  Multiply4/1 -> Product4/2
  [p] -> Product7/2
  Add5/1 -> Product7/1
  Constant3/1 -> Sum3/1
  [beta] -> n-D Lookup Table1/2, CY_da1/2, CY2/2, CY_da20lef/2
  CY1/1 -> Add/2
  [dlef] -> Multiply1/1
  Add4/1 -> Product4/1
  Product5/1 -> [CY_dr30_CY]
  Constant2/1 -> Sum2/1
  [alpha] -> CYp/1
  [bi2vel] -> Product8/2
  Product/1 -> [dCY_lef_1_dlef_25]
  Multiply/1 -> Sum/2
  [dlef] -> Multiply3/1
  Multiply5/1 -> Product5/2
  Sum2/1 -> Product2/2
  [alpha] -> dCY_lef/1, CY/1
  n-D Lookup Table1/1 -> Add1/2
  [beta] -> CY_da20/2, CY1/2
  Add7/1 -> CY_t/1
  Product8/1 -> [CYr_CYp]
  Multiply2/1 -> Sum2/2
  [dlef] -> Multiply2/1
  Add6/1 -> Product8/1
  [alpha] -> n-D Lookup Table/1
  [alpha] -> n-D Lookup Table2/1
  CY_dr30/1 -> Add2/1
  [da] -> Multiply4/1
  [alpha] -> CY_dr30/1, CY3/1
  [dr] -> Multiply5/1
  [alpha] -> dCYr_lef/1
  dCY_da20lef/1 -> Product1/1
  dCYr_lef/1 -> Product2/1
  [beta] -> n-D Lookup Table/2
  Sum/1 -> Product/2
  CY/1 -> dcy,lef/2
  [CY_da20_CY] -> Add7/3
  dCY_lef/1 -> dcy,lef/1
  dCYp_lef/1 -> Product3/1
  CY3/1 -> Add2/2
  CY_da20/1 -> Add/1
  CY_da20lef/1 -> dCY_da20lef/1
  Add1/1 -> dCY_da20lef/3
  CY_da1/1 -> Add1/1
  Multiply1/1 -> Sum1/2
  CY2/1 -> dCY_da20lef/2
  Product3/1 -> Add5/2
  Add3/1 -> Product6/1
  Product2/1 -> Add3/2
  Sum3/1 -> Product3/2
  Multiply3/1 -> Sum3/2
  [alpha] -> dCYp_lef/1
  [CY_dr30_CY] -> Add7/4
  [CYr_CYp] -> Add7/5
  [dCY_lef_1_dlef_25] -> Add7/2
  [CY] -> Add7/1
  Product4/1 -> [CY_da20_CY]
  Product7/1 -> Add6/2
  CYp/1 -> Add5/1
  Alpha/1 -> [alpha]
  beta/1 -> [beta]
  dlef/1 -> [dlef]
  da/1 -> [da]
  dr/1 -> [dr]
  r/1 -> [r]
  bi2vel/1 -> [bi2vel]
  p/1 -> [p]

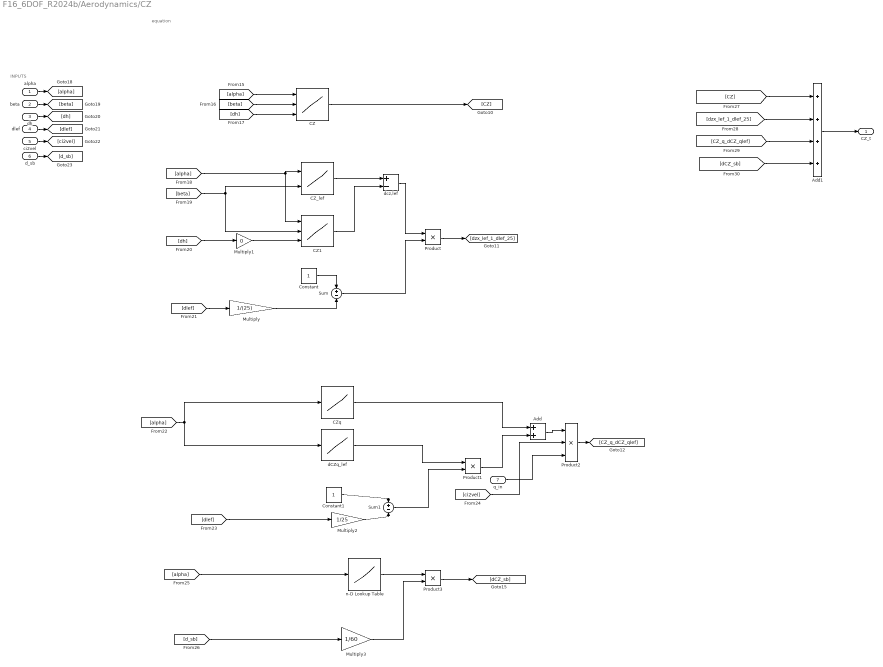
== system F16_6DOF_R2024b/Aerodynamics/CZ ==
  note: INPUTS
  note: equation
  alpha : Inport
  beta : Inport  Port=2
  dh : Inport  Port=3
  dlef : Inport  Port=4
  ci2vel : Inport  Port=5
  d_sb : Inport  Port=6
  q_in : Inport  Port=7
  Add : Sum
  Add1 : Sum  Inputs=4
  CZ : Lookup_n-D  NumberOfTableDimensions=3  BreakpointsForDimension1=AeroBP.CZ.CZ.alpha  BreakpointsForDimension2=AeroBP.CZ.CZ.beta  BreakpointsForDimension3=AeroBP.CZ.CZ.dHT  Table=AeroData.CZ.CZ  ExtrapMethod=Clip  InternalRulePriority=Speed  RndMeth=Simplest
      settings: InputPortMap=u0,u1,u2
  CZ1 : Lookup_n-D  NumberOfTableDimensions=3  BreakpointsForDimension1=AeroBP.CZ.CZ.alpha  BreakpointsForDimension2=AeroBP.CZ.CZ.beta  BreakpointsForDimension3=AeroBP.CZ.CZ.dHT  Table=AeroData.CZ.CZ  ExtrapMethod=Clip  InternalRulePriority=Speed  RndMeth=Simplest
      settings: InputPortMap=u0,u1,u2
  CZ_lef : Lookup_n-D  BreakpointsForDimension1=AeroBP.CZ.CZlef.alpha  BreakpointsForDimension2=AeroBP.CZ.CZlef.beta  BreakpointsForDimension3=[5, 7]  Table=AeroData.CZ.CZlef  ExtrapMethod=Clip  InternalRulePriority=Speed  RndMeth=Simplest
      settings: InputPortMap=u0,u1
  CZq : Lookup_n-D  NumberOfTableDimensions=1  BreakpointsForDimension1=AeroBP.CZ.CZq.alpha  BreakpointsForDimension3=[5, 7]  Table=AeroData.CZ.CZq  ExtrapMethod=Clip  InternalRulePriority=Speed  RndMeth=Simplest
  Constant : Constant
  Constant1 : Constant
  Multiply : Gain  Gain=1/(25)
  Multiply1 : Gain  Gain=0
  Multiply2 : Gain  Gain=1/25
  Multiply3 : Gain  Gain=1/60
  Product : Product
  Product1 : Product
  Product2 : Product  Inputs=3
  Product3 : Product
  Sum : Sum  Inputs=+-
  Sum1 : Sum  Inputs=+-
  dCZq_lef : Lookup_n-D  NumberOfTableDimensions=1  BreakpointsForDimension1=AeroBP.CZ.deltaCZqlef.alpha  BreakpointsForDimension3=[5, 7]  Table=AeroData.CZ.deltaCZqlef  ExtrapMethod=Clip  InternalRulePriority=Speed  RndMeth=Simplest
  dcz,lef : Sum  Inputs=+-
  n-D Lookup Table : Lookup_n-D  NumberOfTableDimensions=1  BreakpointsForDimension1=AeroBP.CZ.deltaCZSB.alpha  BreakpointsForDimension3=[5, 7]  Table=AeroData.CZ.deltaCZSB  ExtrapMethod=Clip  InternalRulePriority=Speed  RndMeth=Simplest
  CZ_t : Outport
  wires:
  Add1/1 -> CZ_t/1
  Multiply3/1 -> Product3/2
  CZ1/1 -> dcz,lef/2
  [dCZ_sb] -> Add1/4
  Multiply2/1 -> Sum1/2
  ci2vel/1 -> [ci2vel]
  Multiply1/1 -> CZ1/3
  [beta] -> CZ_lef/2, CZ1/2
  n-D Lookup Table/1 -> Product3/1
  [alpha] -> CZ1/1, CZ_lef/1
  CZq/1 -> Add/1
  [alpha] -> CZq/1, dCZq_lef/1
  [alpha] -> n-D Lookup Table/1
  d_sb/1 -> [d_sb]
  [dlef] -> Multiply/1
  Product3/1 -> [dCZ_sb]
  Constant1/1 -> Sum1/1
  [beta] -> CZ/2
  Sum/1 -> Product/2
  [CZ] -> Add1/1
  [alpha] -> CZ/1
  dCZq_lef/1 -> Product1/1
  [dzx_lef_1_dlef_25] -> Add1/2
  [d_sb] -> Multiply3/1
  [ci2vel] -> Product2/2
  [CZ_q_dCZ_qlef] -> Add1/3
  Product2/1 -> [CZ_q_dCZ_qlef]
  dh/1 -> [dh]
  [dh] -> CZ/3
  CZ/1 -> [CZ]
  Product/1 -> [dzx_lef_1_dlef_25]
  dlef/1 -> [dlef]
  Multiply/1 -> Sum/2
  [dh] -> Multiply1/1
  CZ_lef/1 -> dcz,lef/1
  Constant/1 -> Sum/1
  dcz,lef/1 -> Product/1
  beta/1 -> [beta]
  Add/1 -> Product2/1
  [dlef] -> Multiply2/1
  Sum1/1 -> Product1/2
  Product1/1 -> Add/2
  alpha/1 -> [alpha]
  q_in/1 -> Product2/3

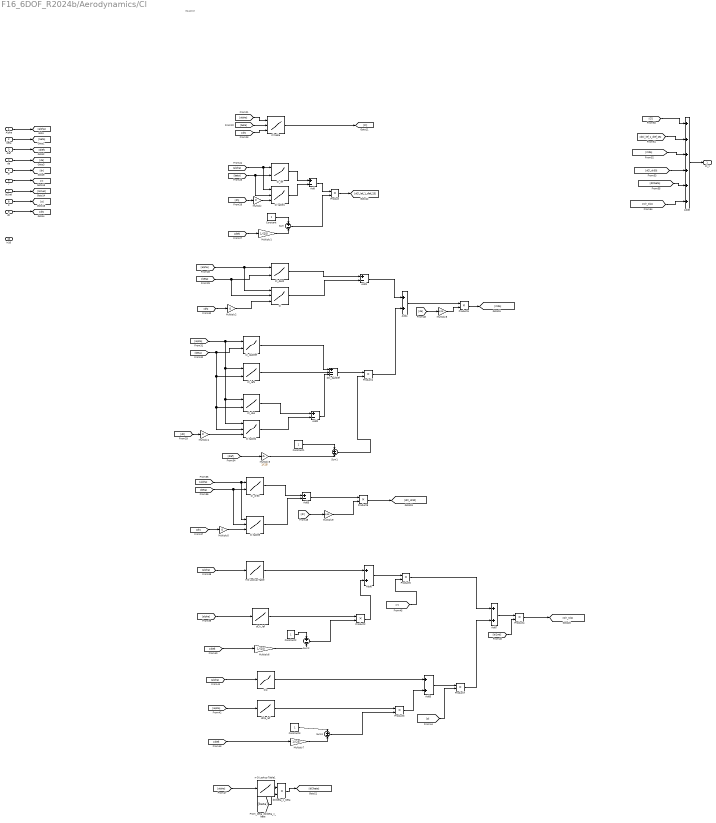
== system F16_6DOF_R2024b/Aerodynamics/Cl ==
  note: equation
  Alpha : Inport
  beta : Inport  Port=2
  dlef : Inport  Port=3
  da : Inport  Port=4
  dr : Inport  Port=5
  r : Inport  Port=6
  bi2vel : Inport  Port=7
  p : Inport  Port=8
  dh : Inport  Port=9
  In10 : Inport  Port=10
  Add{,1..3} (4 alike) : Sum  Inputs=+-
  Add{4..7} (4 alike) : Sum
  Add8 : Sum  Inputs=6
  Cl : Lookup_n-D  NumberOfTableDimensions=3  BreakpointsForDimension1=AeroBP.Cl.Cl.alpha  BreakpointsForDimension2=AeroBP.Cl.Cl.beta  BreakpointsForDimension3=AeroBP.Cl.Cl.dHT  Table=AeroData.Cl.Cl  ExtrapMethod=Clip  InternalRulePriority=Speed  RndMeth=Simplest
      settings: InputPortMap=u0,u1,u2
  Cl table{,1..3} (4 alike) : Lookup_n-D  NumberOfTableDimensions=3  BreakpointsForDimension1=AeroBP.Cl.Cl.alpha  BreakpointsForDimension2=AeroBP.Cl.Cl.beta  BreakpointsForDimension3=AeroBP.Cl.Cl.dHT  Table=AeroData.Cl.Cl  ExtrapMethod=Clip  InternalRulePriority=Speed  RndMeth=Simplest
      settings: InputPortMap=u0,u1,u2
  Cl_da1 : Lookup_n-D  BreakpointsForDimension1=AeroBP.Cl.Clda20.alpha  BreakpointsForDimension2=AeroBP.Cl.Clda20.beta  BreakpointsForDimension3=[5, 7]  Table=AeroData.Cl.Clda20  ExtrapMethod=Clip  InternalRulePriority=Speed  RndMeth=Simplest
      settings: InputPortMap=u0,u1
  Cl_da20 : Lookup_n-D  BreakpointsForDimension1=AeroBP.Cl.Clda20.alpha  BreakpointsForDimension2=AeroBP.Cl.Clda20.beta  BreakpointsForDimension3=[5, 7]  Table=AeroData.Cl.Clda20  ExtrapMethod=Clip  InternalRulePriority=Speed  RndMeth=Simplest
      settings: InputPortMap=u0,u1
  Cl_da20lef : Lookup_n-D  BreakpointsForDimension1=AeroBP.Cl.Clda20lef.alpha  BreakpointsForDimension2=AeroBP.Cl.Clda20lef.beta  BreakpointsForDimension3=[5, 7]  Table=AeroData.Cl.Clda20lef  ExtrapMethod=Clip  InternalRulePriority=Speed  RndMeth=Simplest
      settings: InputPortMap=u0,u1
  Cl_dr30 : Lookup_n-D  BreakpointsForDimension1=AeroBP.Cl.Cldr30.alpha  BreakpointsForDimension2=AeroBP.Cl.Cldr30.beta  BreakpointsForDimension3=[5, 7]  Table=AeroData.Cl.Cldr30  ExtrapMethod=Clip  InternalRulePriority=Speed  RndMeth=Simplest
      settings: InputPortMap=u0,u1
  Cl_lef : Lookup_n-D  BreakpointsForDimension1=AeroBP.Cl.Cllef.alpha  BreakpointsForDimension2=AeroBP.Cl.Cllef.beta  BreakpointsForDimension3=[5, 7]  Table=AeroData.Cl.Cllef  ExtrapMethod=Clip  InternalRulePriority=Speed  RndMeth=Simplest
      settings: InputPortMap=u0,u1
  Cl_lef1 : Lookup_n-D  BreakpointsForDimension1=AeroBP.Cl.Cllef.alpha  BreakpointsForDimension2=AeroBP.Cl.Cllef.beta  BreakpointsForDimension3=[5, 7]  Table=AeroData.Cl.Cllef  ExtrapMethod=Clip  InternalRulePriority=Speed  RndMeth=Simplest
      settings: InputPortMap=u0,u1
  Clp : Lookup_n-D  NumberOfTableDimensions=1  BreakpointsForDimension1=AeroBP.Cl.Clp.alpha  BreakpointsForDimension3=[5, 7]  Table=AeroData.Cl.Clp  ExtrapMethod=Clip  InternalRulePriority=Speed  RndMeth=Simplest
  Constant{,1..3} (4 alike) : Constant
  Multiply{,2,4..5} (4 alike) : Gain  Gain=0
  Multiply{1,3,6..7} (4 alike) : Gain  Gain=1/(25)
  Multiply8 : Gain  Gain=1/20
  Multiply9 : Gain  Gain=1/30
  Product{,1..8} (9 alike) : Product
  Sum{,1..3} (4 alike) : Sum  Inputs=+-
  dCl_da20lef : Sum  Inputs=+--
  dClbeta_x_beta : Product
  dClp_lef : Lookup_n-D  NumberOfTableDimensions=1  BreakpointsForDimension1=AeroBP.Cl.deltaClplef.alpha  BreakpointsForDimension3=[5, 7]  Table=AeroData.Cl.deltaClplef  ExtrapMethod=Clip  InternalRulePriority=Speed  RndMeth=Simplest
  dClr_lef : Lookup_n-D  NumberOfTableDimensions=1  BreakpointsForDimension1=AeroBP.Cl.deltaClrlef.alpha  BreakpointsForDimension3=[5, 7]  Table=AeroData.Cl.deltaClrlef  ExtrapMethod=Clip  InternalRulePriority=Speed  RndMeth=Simplest
  n-D Lookup Table : Lookup_n-D  NumberOfTableDimensions=1  BreakpointsForDimension1=AeroBP.Cl.Clr.alpha  BreakpointsForDimension3=[5, 7]  Table=AeroData.Cl.Clr  ExtrapMethod=Clip  InternalRulePriority=Speed  RndMeth=Simplest
  n-D Lookup Table1 : Lookup_n-D  NumberOfTableDimensions=1  BreakpointsForDimension1=AeroBP.Cl.deltaClBeta.alpha  BreakpointsForDimension3=[5, 7]  Table=AeroData.Cl.deltaClBeta  ExtrapMethod=Clip  InternalRulePriority=Speed  RndMeth=Simplest
  Cl_t : Outport
  wires:
  [beta] -> Cl table1/2, Cl_lef/2
  [beta] -> Cl_da20lef/2, Cl table2/2, Cl_da1/2, Cl_lef1/2
  Multiply1/1 -> Sum/2
  Product8/1 -> [dCl_dr30]
  Multiply8/1 -> Product6/2
  Sum3/1 -> Product3/2
  [alpha] -> n-D Lookup Table1/1
  [beta] -> Cl_da20/2, Cl/2
  Multiply3/1 -> Sum1/2
  Cl table2/1 -> Add2/2
  [r] -> Product5/2
  [dh] -> Multiply2/1
  [alpha] -> Cl_da20lef/1, Cl table2/1, Cl_da1/1, Cl_lef1/1
  [da] -> Multiply8/1
  Multiply2/1 -> Cl/3
  Cl table/1 -> [Cl]
  [beta] -> Cl table/2
  Product/1 -> [dCl_lef_1_dlef_25]
  Add/1 -> Product/1
  [alpha] -> Clp/1
  Multiply6/1 -> Sum2/2
  [alpha] -> Cl table/1
  Constant/1 -> Sum/1
  Multiply4/1 -> Cl table2/3
  Cl_lef/1 -> Add/1
  [dh] -> Cl table/3
  Add2/1 -> dCl_da20lef/3
  [alpha] -> Cl table1/1, Cl_lef/1
  [alpha] -> n-D Lookup Table/1
  Add3/1 -> Product8/1
  [alpha] -> Cl table3/1, Cl_dr30/1
  Product3/1 -> Add5/2
  dCl_da20lef/1 -> Product1/1
  [Clr_Clp] -> Add8/6
  dClr_lef/1 -> Product2/1
  Cl table3/1 -> Add3/2
  [dlef] -> Multiply6/1
  Constant3/1 -> Sum3/1
  dClp_lef/1 -> Product3/1
  Add5/1 -> Product7/1
  [bi2vel] -> Product4/2
  Product4/1 -> [Clr_Clp]
  Product2/1 -> Add6/2
  [dCl_lef_1_dlef_25] -> Add8/2
  Sum2/1 -> Product2/2
  [p] -> Product7/2
  Sum/1 -> Product/2
  Multiply7/1 -> Sum3/2
  [dh] -> Multiply/1
  [beta] -> Cl table3/2, Cl_dr30/2
  [dClbeta] -> Add8/5
  Sum1/1 -> Product1/2
  Multiply9/1 -> Product8/2
  Cl_lef1/1 -> dCl_da20lef/2
  Cl/1 -> Add1/2
  Cl_da1/1 -> Add2/1
  Cl_da20lef/1 -> dCl_da20lef/1
  Constant1/1 -> Sum1/1
  [alpha] -> Cl_da20/1, Cl/1
  Cl_da20/1 -> Add1/1
  n-D Lookup Table/1 -> Add6/1
  Add6/1 -> Product5/1
  Product7/1 -> Add7/2
  [dh] -> Multiply5/1
  [dlef] -> Multiply1/1
  [alpha] -> dClr_lef/1
  [Clda] -> Add8/3
  [Cl] -> Add8/1
  Add8/1 -> Cl_t/1
  Clp/1 -> Add5/1
  Add7/1 -> Product4/1
  Constant2/1 -> Sum2/1
  Cl table1/1 -> Add/2
  [alpha] -> dClp_lef/1
  [dlef] -> Multiply3/1
  Multiply5/1 -> Cl table3/3
  Cl_dr30/1 -> Add3/1
  [dlef] -> Multiply7/1
  Product5/1 -> Add7/1
  [dh] -> Multiply4/1
  Multiply/1 -> Cl table1/3
  Add1/1 -> Add4/1
  [dr] -> Multiply9/1
  Add4/1 -> Product6/1
  Product6/1 -> [Clda]
  Product1/1 -> Add4/2
  r/1 -> [r]
  p/1 -> [p]
  dlef/1 -> [dlef]
  dr/1 -> [dr]
  da/1 -> [da]
  beta/1 -> [beta]
  Alpha/1 -> [alpha]
  bi2vel/1 -> [bi2vel]
  [dCl_dr30] -> Add8/4
  dh/1 -> [dh]
  n-D Lookup Table1/1 -> dClbeta_x_beta/1
  [beta] -> dClbeta_x_beta/2
  dClbeta_x_beta/1 -> [dClbeta]

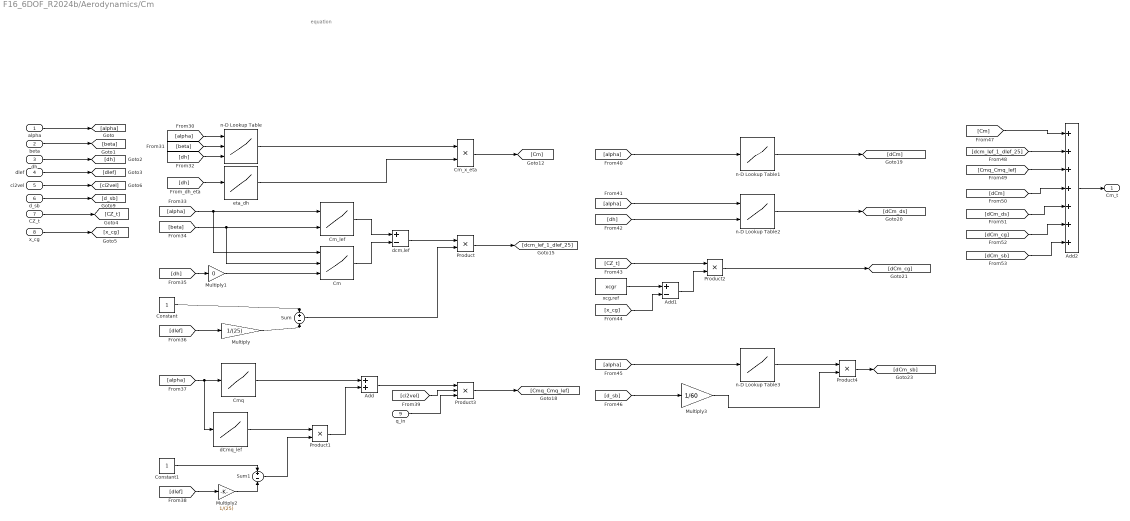
== system F16_6DOF_R2024b/Aerodynamics/Cm ==
  note: equation
  alpha : Inport
  beta : Inport  Port=2
  dh : Inport  Port=3
  dlef : Inport  Port=4
  ci2vel : Inport  Port=5
  d_sb : Inport  Port=6
  CZ_t : Inport  Port=7
  x_cg : Inport  Port=8
  q_in : Inport  Port=9
  Add : Sum
  Add1 : Sum  Inputs=+-
  Add2 : Sum  Inputs=+++++++
  Cm : Lookup_n-D  NumberOfTableDimensions=3  BreakpointsForDimension1=AeroBP.Cm.Cm.alpha  BreakpointsForDimension2=AeroBP.Cm.Cm.beta  BreakpointsForDimension3=AeroBP.Cm.Cm.dHT  Table=AeroData.Cm.Cm  ExtrapMethod=Clip  InternalRulePriority=Speed  RndMeth=Simplest
      settings: InputPortMap=u0,u1,u2
  Cm_lef : Lookup_n-D  BreakpointsForDimension1=AeroBP.Cm.Cmlef.alpha  BreakpointsForDimension2=AeroBP.Cm.Cmlef.beta  BreakpointsForDimension3=[5, 7]  Table=AeroData.Cm.Cmlef  ExtrapMethod=Clip  InternalRulePriority=Speed  RndMeth=Simplest
      settings: InputPortMap=u0,u1
  Cm_x_eta : Product
  Cmq : Lookup_n-D  NumberOfTableDimensions=1  BreakpointsForDimension1=AeroBP.Cm.Cmq.alpha  BreakpointsForDimension3=[5, 7]  Table=AeroData.Cm.Cmq  ExtrapMethod=Clip  InternalRulePriority=Speed  RndMeth=Simplest
  Constant : Constant
  Constant1 : Constant
  Multiply : Gain  Gain=1/(25)
  Multiply1 : Gain  Gain=0
  Multiply2 : Gain  Gain=1/(25)
  Multiply3 : Gain  Gain=1/60
  Product{,1..2,4} (4 alike) : Product
  Product3 : Product  Inputs=3
  Sum : Sum  Inputs=+-
  Sum1 : Sum  Inputs=+-
  dCmq_lef : Lookup_n-D  NumberOfTableDimensions=1  BreakpointsForDimension1=AeroBP.Cm.deltaCmqlef.alpha  BreakpointsForDimension3=[5, 7]  Table=AeroData.Cm.deltaCmqlef  ExtrapMethod=Clip  InternalRulePriority=Speed  RndMeth=Simplest
  dcm,lef : Sum  Inputs=+-
  eta_dh : Lookup_n-D  NumberOfTableDimensions=1  BreakpointsForDimension1=AeroBP.Cm.n_dHT.dHT  Table=AeroData.Cm.n_dHT  ExtrapMethod=Clip  InternalRulePriority=Speed  RndMeth=Simplest
  n-D Lookup Table : Lookup_n-D  NumberOfTableDimensions=3  BreakpointsForDimension1=AeroBP.Cm.Cm.alpha  BreakpointsForDimension2=AeroBP.Cm.Cm.beta  BreakpointsForDimension3=AeroBP.Cm.Cm.dHT  Table=AeroData.Cm.Cm  ExtrapMethod=Clip  InternalRulePriority=Speed  RndMeth=Simplest
      settings: InputPortMap=u0,u1,u2
  n-D Lookup Table1 : Lookup_n-D  NumberOfTableDimensions=1  BreakpointsForDimension1=AeroBP.Cm.deltaCm.alpha  BreakpointsForDimension3=[5, 7]  Table=AeroData.Cm.deltaCm  ExtrapMethod=Clip  InternalRulePriority=Speed  RndMeth=Simplest
  n-D Lookup Table2 : Lookup_n-D  BreakpointsForDimension1=AeroBP.Cm.deltaCmds.alpha  BreakpointsForDimension2=AeroBP.Cm.deltaCmds.dHT  BreakpointsForDimension3=[5, 7]  Table=AeroData.Cm.deltaCmds  ExtrapMethod=Clip  InternalRulePriority=Speed  RndMeth=Simplest
      settings: InputPortMap=u0,u1
  n-D Lookup Table3 : Lookup_n-D  NumberOfTableDimensions=1  BreakpointsForDimension1=AeroBP.Cm.deltaCmSB.alpha  BreakpointsForDimension3=[5, 7]  Table=AeroData.Cm.deltaCmSB  ExtrapMethod=Clip  InternalRulePriority=Speed  RndMeth=Simplest
  xcg,ref : Constant  Value=xcgr
  Cm_t : Outport
  wires:
  Product2/1 -> [dCm_cg]
  [ci2vel] -> Product3/2
  [d_sb] -> Multiply3/1
  Product3/1 -> [Cmq_Cmq_lef]
  n-D Lookup Table3/1 -> Product4/1
  n-D Lookup Table2/1 -> [dCm_ds]
  [alpha] -> n-D Lookup Table3/1
  [dcm_lef_1_dlef_25] -> Add2/2
  Multiply1/1 -> Cm/3
  [CZ_t] -> Product2/1
  Multiply3/1 -> Product4/2
  Product1/1 -> Add/2
  [dh] -> Multiply1/1
  [beta] -> Cm_lef/2, Cm/2
  [alpha] -> n-D Lookup Table1/1
  [x_cg] -> Add1/2
  [alpha] -> Cmq/1, dCmq_lef/1
  Multiply/1 -> Sum/2
  [dlef] -> Multiply2/1
  [Cm] -> Add2/1
  xcg,ref/1 -> Add1/1
  Cm/1 -> dcm,lef/2
  Constant1/1 -> Sum1/1
  [Cmq_Cmq_lef] -> Add2/3
  Cm_lef/1 -> dcm,lef/1
  n-D Lookup Table1/1 -> [dCm]
  Sum/1 -> Product/2
  [alpha] -> n-D Lookup Table2/1
  dcm,lef/1 -> Product/1
  Constant/1 -> Sum/1
  Add2/1 -> Cm_t/1
  [beta] -> n-D Lookup Table/2
  [alpha] -> Cm_lef/1, Cm/1
  Sum1/1 -> Product1/2
  Multiply2/1 -> Sum1/2
  [dh] -> n-D Lookup Table2/2
  [dh] -> n-D Lookup Table/3
  [dCm] -> Add2/4
  Product/1 -> [dcm_lef_1_dlef_25]
  [alpha] -> n-D Lookup Table/1
  [dCm_cg] -> Add2/6
  [dCm_ds] -> Add2/5
  [dlef] -> Multiply/1
  Add1/1 -> Product2/2
  Add/1 -> Product3/1
  [dCm_sb] -> Add2/7
  ci2vel/1 -> [ci2vel]
  dh/1 -> [dh]
  alpha/1 -> [alpha]
  dlef/1 -> [dlef]
  d_sb/1 -> [d_sb]
  beta/1 -> [beta]
  CZ_t/1 -> [CZ_t]
  x_cg/1 -> [x_cg]
  q_in/1 -> Product3/3
  n-D Lookup Table/1 -> Cm_x_eta/1
  eta_dh/1 -> Cm_x_eta/2
  [dh] -> eta_dh/1
  Cm_x_eta/1 -> [Cm]
  Product4/1 -> [dCm_sb]
  dCmq_lef/1 -> Product1/1
  Cmq/1 -> Add/1
